simulink model "CurrentLoopTest"  (R2026b)
settings: Solver=ode4  StopTime=fixtureCfg.Duration  FixedStep=experimentCfg.Step
PostLoadFcn:
  | addpath(fullfile(fileparts(fileparts(fileparts(fileparts(fileparts(get_param(bdroot,'FileName')))))),'docs','scripts'));initialize_motor_paths();initialize_motor_model(bdroot);
model workspace (MAT data in the model file):
  currentCfg.Ts = 0.0001
  currentCfg.BandwidthHz = 500
  currentCfg.Kpd = 3.14159265359
  currentCfg.Kpq = 3.76991118431
  currentCfg.Kid = 1570.79632679
  currentCfg.Kiq = 1570.79632679
  currentCfg.Kaw = 1000
  deadtimeCfg.DeadTime = 2e-06
  deadtimeCfg.DeviceDrop = 0
  deadtimeCfg.CurrentBlend = 0.1
  deadtimeCfg.ModelEnable = 0
  deadtimeCfg.CompensationEnable = 0
  deadtimeCfg.CompensationScale = 1
  deadtimeCfg.SwitchingStep = 1e-07
  experimentCfg.Step = 5e-06
  experimentCfg.LogTs = 0.0001
  experimentCfg.Duration = 1.5
  experimentCfg.Mode = 2
  experimentCfg.UseInverter = 1
  experimentCfg.UseTiming = 1
  experimentCfg.UseMechanical = 1
  experimentCfg.ImposedElectricalSpeed = 0
  experimentCfg.IdReference = 0
  experimentCfg.IqReference = 2
  experimentCfg.IqInitial = 0
  experimentCfg.SpeedReference = 40
  experimentCfg.SpeedInitial = 0
  experimentCfg.PositionReference = 1
  experimentCfg.PositionInitial = 0
  experimentCfg.CommandTime = 0.05
  experimentCfg.LoadTorque = 0.1
  experimentCfg.LoadTime = 0.35
  experimentCfg.Enable = 1
  experimentCfg.Reset = 0
  feedforwardCfg.Enable = 0
  feedforwardCfg.ParameterScale = 1
  fixtureCfg.Ts = 0.0001
  fixtureCfg.Duration = 0.03
  fixtureCfg.SolverStep = 5e-06
  fixtureCfg.IdReference = 0
  fixtureCfg.IqReference = 2
  fixtureCfg.CommandTime = 0.003
  fixtureCfg.ElectricalSpeed = 0
  fixtureCfg.Enable = 1
  fixtureCfg.Reset = 0
  fixtureCfg.Inputs = [0 0 0 0 0 0 0 0 0 0 0 0 ... (1505 elements, 301x5)]
  inverterCfg.Vdc = 48
  inverterCfg.MinDuty = 0.02
  inverterCfg.PwmTs = 0.0001
  inverterCfg.LinearLimit = 26.6043004043
  motionCfg.Ts = 0.001
  motionCfg.NaturalFrequency = 20
  motionCfg.Damping = 0.9
  motionCfg.Kt = 0.21
  motionCfg.Kp = 0.0852380952381
  motionCfg.Ki = 0.952380952381
  motionCfg.Kaw = 20
  motionCfg.PositionKp = 8
  motionCfg.SpeedLimit = 80
  motionCfg.AccelerationLimit = 200
  motionCfg.CurrentLimit = 8
  pmsmCfg.Rs = 0.5
  pmsmCfg.Ld = 0.001
  pmsmCfg.Lq = 0.0012
  pmsmCfg.Flux = 0.035
  pmsmCfg.PolePairs = 4
  pmsmCfg.J = 0.0005
  pmsmCfg.B = 0.0001
  pmsmCfg.Id0 = 0
  pmsmCfg.Iq0 = 0
  pmsmCfg.Speed0 = 0
  pmsmCfg.Position0 = 0
  testStim.time = []
  testStim.signals.values = [0 0 0 0 0 0 0 0 0 0 0 0 ... (1505 elements, 301x5)]
  testStim.signals.dimensions = 5
  timingCfg.Ts = 0.0001
  timingCfg.FeedbackTicks = 1
  timingCfg.ActuationTicks = 1
libraries: CurrentControl x2, PMSMPlant x1
settings Model: Creator=24322  LastModifiedBy=24322

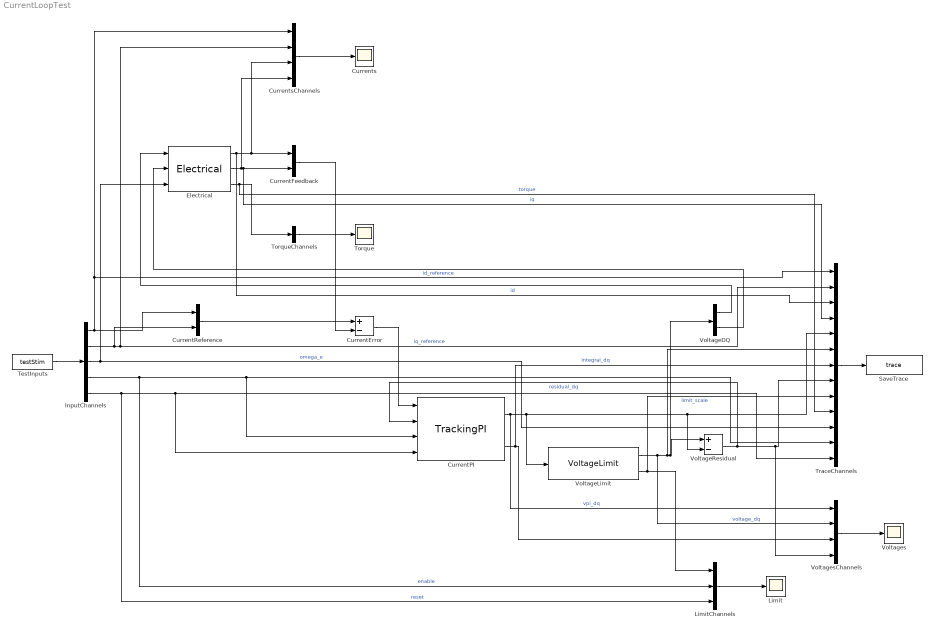
== system CurrentLoopTest ==
  CurrentError : Sum  Inputs=+-
  CurrentFeedback : Mux  Inputs=2
  CurrentPI : CurrentControl/TrackingPI  SystemSampleTime=-1  VariantActivationTime=update diagram  EmptyChoice=off  PassThrough=off  PassThroughVariantControl=(default)  EmptyChoiceVariantControl=(default)  AllowFlexibleInterface=on  Latency=0  AutoFrameSizeCalculation=off
  CurrentReference : Mux  Inputs=2
  Currents : Scope
      settings: Title=Currents  YLabel=A
  CurrentsChannels : Mux
  Electrical : PMSMPlant/Electrical  SystemSampleTime=-1  VariantActivationTime=update diagram  EmptyChoice=off  PassThrough=off  PassThroughVariantControl=(default)  EmptyChoiceVariantControl=(default)  AllowFlexibleInterface=on  Latency=0  AutoFrameSizeCalculation=off
  InputChannels : Demux  Outputs=5
  Limit : Scope
      settings: Title=Limit  YLabel=1
  LimitChannels : Mux  Inputs=3
  SaveTrace : ToWorkspace  VariableName=trace  SaveFormat=Structure With Time  SampleTime=experimentCfg.LogTs
  TestInputs : FromWorkspace  VariableName=testStim  SampleTime=currentCfg.Ts  Interpolate=off  OutputAfterFinalValue=Holding final value
  Torque : Scope
      settings: Title=Torque  YLabel=N*m
  TorqueChannels : Mux  Inputs=1
  TraceChannels : Mux  Inputs=13
  VoltageDQ : Demux  Outputs=2
  VoltageLimit : CurrentControl/VoltageLimit  SystemSampleTime=-1  VariantActivationTime=update diagram  EmptyChoice=off  PassThrough=off  PassThroughVariantControl=(default)  EmptyChoiceVariantControl=(default)  AllowFlexibleInterface=on  Latency=0  AutoFrameSizeCalculation=off
  VoltageResidual : Sum  Inputs=+-
  Voltages : Scope
      settings: Title=Voltages  YLabel=V
  VoltagesChannels : Mux
  wires:
  TorqueChannels/1 -> Torque/1
  LimitChannels/1 -> Limit/1
  VoltagesChannels/1 -> Voltages/1
  CurrentsChannels/1 -> Currents/1
  Electrical/3 -> TraceChannels/10, TorqueChannels/1  "torque"
  VoltageLimit/2 -> TraceChannels/9, LimitChannels/1  "limit_scale"
  CurrentPI/2 -> TraceChannels/7, VoltagesChannels/3  "integral_dq"
  TraceChannels/1 -> SaveTrace/1
  InputChannels/3 -> Electrical/3, TraceChannels/11  "omega_e"
  VoltageDQ/2 -> Electrical/2
  VoltageDQ/1 -> Electrical/1
  VoltageLimit/1 -> VoltageResidual/1, VoltageDQ/1, TraceChannels/6, VoltagesChannels/2  "voltage_dq"
  CurrentPI/1 -> TraceChannels/5, VoltageResidual/2, VoltageLimit/1, VoltagesChannels/1  "vpi_dq"
  InputChannels/5 -> CurrentPI/4, TraceChannels/13, LimitChannels/3  "reset"
  InputChannels/4 -> CurrentPI/3, TraceChannels/12, LimitChannels/2  "enable"
  VoltageResidual/1 -> TraceChannels/8, VoltagesChannels/4, CurrentPI/2  "residual_dq"
  CurrentError/1 -> CurrentPI/1
  CurrentFeedback/1 -> CurrentError/2
  CurrentReference/1 -> CurrentError/1
  Electrical/2 -> CurrentFeedback/2, TraceChannels/4, CurrentsChannels/4  "iq"
  Electrical/1 -> CurrentFeedback/1, CurrentsChannels/3, TraceChannels/3  "id"
  InputChannels/2 -> CurrentsChannels/2, TraceChannels/2, CurrentReference/2  "iq_reference"
  InputChannels/1 -> CurrentsChannels/1, TraceChannels/1, CurrentReference/1  "id_reference"
  TestInputs/1 -> InputChannels/1
